simulink model "speedgoat_IO397_RCP_BLDC_openloop"  (R2025b)
settings: Solver=FixedStepDiscrete  StartTime=0.0  StopTime=inf  RelTol=1e-3
PreLoadFcn:
  | Ts = 0.001;
  | FPGA_Frequency = 75000000;
InitFcn:
  | load speedgoat_IO397_RCP_OpenLoop_Initialize.mat;
values from neighbouring files (symbols this model uses):
  motor =     [speedgoat_IO397_RCP_OpenLoop_Initialize.mat]
  target =     [speedgoat_IO397_RCP_OpenLoop_Initialize.mat]
undefined symbols (not defined in the file or in its folder): bit, DiscIntNeverNeededParam, IO397, Pull, pull, up
libraries: mcbcontrolslib x4, mcbpositiondecoderlib x3, c2837xDlib x2, c2802xlib x2, speedgoatlib_fpga_dio x1, speedgoatlib_fpga_analog_io x1, speedgoatlib_fpga_pwm x1, speedgoatlib_fpga_quadrature x1, speedgoatlib_fpga x1
settings Model: SimulationMode=external  ExtModeEnableFloating=off  Creator=simon.beck  LastModifiedBy=PattarapolSangaroon
settings SolverCC: ConcurrentTasks=on  PositivePriorityOrder=on  MaxZcPerStep=1.0
settings DataIOCC: SaveFormat=StructureWithTime
settings OptimizationCC: BlockReduction=off  OptimizeBlockIOStorage=off  BufferReuse=off  ReuseModelBlockBuffer=off
settings DebuggingCC: UnderspecifiedInitializationDetection=Classic  MergeDetectMultiDrivingBlocksExec=none  TasksWithSamePriorityMsg=none
settings HardwareCC: ProdBitPerLong=64.0  ProdLongLongMode=on  ProdHWDeviceType=Intel->x86-64 (Linux 64)
settings ModelReferenceCC: EnableRefExpFcnMdlSchedulingChecks=on  PropagateSignalLabelsOutOfModel=off
settings RTWCC: SystemTargetFile=speedgoat.tlc  TemplateMakefile=slrealtime_default_tmf  Toolchain=Simulink Real-Time Toolchain  BuildConfiguration=Faster Runs  CodeExecutionProfiling=on  TargetLang=C++  GPUComputeCapability=3.5  DLArmComputeVersion=19.05  Description=Speedgoat Real-Time Target Machine
settings SimulinkRealTimeTargetCC: SLRTFileLogMaxRuns=1.0  ExtModeMaxTrigDuration=10.0  ExtModeStaticAllocSize=1000000.0  ExtModeTransport=0.0  MultiwordLength=2048.0  DynamicStringBufferSize=256.0  PreserveMATLABNamespacesInGeneratedCode=on  SubcomponentCodeInterfacePackaging=Reusable function  InstructionSetFMA=off  LogToMDFFile=off

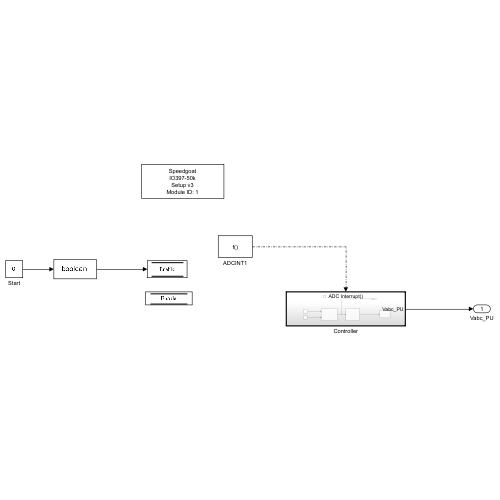
[thumbnail: Simulink's stored preview of the top-level diagram]
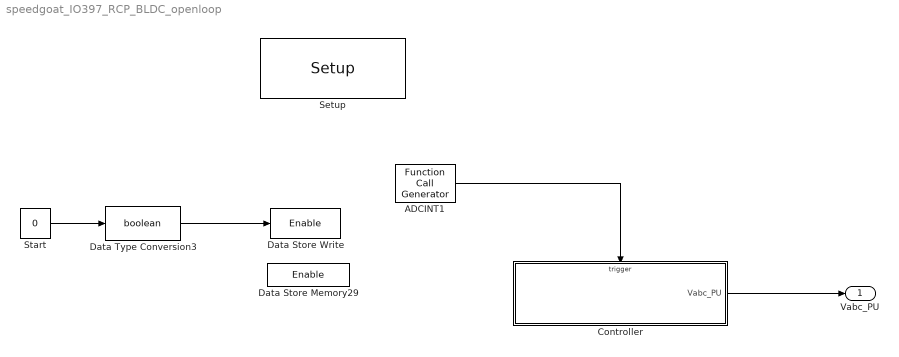
== system speedgoat_IO397_RCP_BLDC_openloop ==
  ADCINT1 : FunctionCallGenerator  SampleTime=Ts
  Controller : Subsystem
  Data Store Memory29 : DataStoreMemory  DataStoreName=Enable  ShowAdditionalParam=off  OutDataTypeStr=boolean
  Data Store Write : DataStoreWrite  DataStoreName=Enable  IndexOptions=Index vector (dialog)  Indices=1  OutputSizes=1
  Data Type Conversion3 : DataTypeConversion  OutDataTypeStr=boolean  RndMeth=Simplest  SaturateOnIntegerOverflow=off
  Setup : speedgoatlib_fpga/Setup/Setup  board=IO397-50k  id=1  pciSlot=-1  device_id=1  bitstreamFilePath=C:\ProgramData\Speedgoat\bitstreams\io_configuration_package\R2025b\io397  bitstreamFile=speedgoat_IO397_RCP.mat  fpgaFreq=75000000  enableDma=off  rearEnb_1=off  rearIO_1=None  rearEnb_2=off  rearIO_2=None  ProgSpiFlash=off  ProgBPIFlash=off  useFpgaDmaController=off  dmaStopOnOverload=on  dmaModeSequential=on  dmaModeParallel=off  dmaTrigFixTime=on  dmaTrigA2B=off  dmaTriggerSourceSel=0  PullRPort15=pull-up 3.3V  PullRPort31=pull-up 3.3V  PullRPort47=pull-up 3.3V  PullRPort63=pull-up 3.3V  diffLineTermination_1=on  diffLineTermination_2=on  diffLineTermination_3=on  diffLineTermination_4=on  diffLineTermination_5=on  diffLineTermination_6=on  diffLineTermination_7=on  diffLineTermination_8=on  diffLineTermination_9=on  diffLineTermination_10=on  diffLineTermination_11=on  diffLineTermination_12=on  diffLineTermination_13=on  diffLineTermination_14=on  diffLineTermination_15=on  diffLineTermination_16=on  diffLineTermination_17=on  diffLineTermination_18=on  diffLineTermination_19=on  diffLineTermination_20=on  diffLineTermination_21=on  diffLineTermination_22=on  diffLineTermination_23=on  diffLineTermination_24=on  diffLineTermination_25=on  diffLineTermination_26=on  diffLineTermination_27=on  diffLineTermination_28=on  diffLineTermination_29=on  diffLineTermination_30=on  diffLineTermination_31=on  diffLineTermination_32=on  ioVoltageDropDown1=3.3V  pullResistorDropDown1_1=Pull-up  pullResistorDropDown1_2=Pull-up  pullResistorDropDown1_3=Pull-up  pullResistorDropDown1_4=Pull-up  pullResistorDropDown1_5=Pull-up  pullResistorDropDown1_6=Pull-up  pullResistorDropDown1_7=Pull-up  pullResistorDropDown1_8=Pull-up  ttlIsImplementedCheckBox1=off  pullResistorDropDown2=Pull-up  ioVoltageDropDown2=3.3V  ttlIsImplementedCheckBox2=off  pullResistorDropDown3=Pull-up  ioVoltageDropDown3=3.3V  ttlIsImplementedCheckBox3=off  pullResistorDropDown4=Pull-up  ioVoltageDropDown4=3.3V  ttlIsImplementedCheckBox4=off  pullResistorDropDown5=Pull-up  ioVoltageDropDown5=3.3V  ttlIsImplementedCheckBox5=off  pullResistorDropDown6=Pull-up  ioVoltageDropDown6=3.3V  ttlIsImplementedCheckBox6=off  pullResistorDropDown7=Pull-up  ioVoltageDropDown7=3.3V  ttlIsImplementedCheckBox7=off  pullResistorDropDown8=Pull-up  ioVoltageDropDown8=3.3V  ttlIsImplementedCheckBox8=off  terminationCheckBox1=off  terminationCheckBox2=off  terminationCheckBox3=off  terminationCheckBox4=off  diffIsImplementedCheckBox1=off  terminationCheckBox5=off  terminationCheckBox6=off  terminationCheckBox7=off  terminationCheckBox8=off  diffIsImplementedCheckBox2=off  terminationCheckBox9=off  terminationCheckBox10=off  terminationCheckBox11=off  terminationCheckBox12=off  diffIsImplementedCheckBox3=off  terminationCheckBox13=off  terminationCheckBox14=off  terminationCheckBox15=off  terminationCheckBox16=off  diffIsImplementedCheckBox4=off  terminationCheckBox17=off  terminationCheckBox18=off  terminationCheckBox19=off  terminationCheckBox20=off  diffIsImplementedCheckBox5=off  terminationCheckBox21=off  terminationCheckBox22=off  terminationCheckBox23=off  terminationCheckBox24=off  diffIsImplementedCheckBox6=off  terminationCheckBox25=off  terminationCheckBox26=off  terminationCheckBox27=off  terminationCheckBox28=off  diffIsImplementedCheckBox7=off  terminationCheckBox29=off  terminationCheckBox30=off  terminationCheckBox31=off  terminationCheckBox32=off  diffIsImplementedCheckBox8=off  PullRPort0_1=pull-up  VioPort0_1=3.3V  PullRPort1_1=pull-up  VioPort1_1=3.3V  PullRPort2_1=pull-up  VioPort2_1=3.3V  PullRPort3_1=pull-up  VioPort3_1=3.3V  PullRPort4_1=pull-up  VioPort4_1=3.3V  PullRPort5_1=pull-up  VioPort5_1=3.3V  PullRPort6_1=pull-up  VioPort6_1=3.3V  diffLineTermination_rear1_1=on  diffLineTermination_rear1_2=on  diffLineTermination_rear1_3=on  diffLineTermination_rear1_4=on  diffLineTermination_rear1_5=on  diffLineTermination_rear1_6=on  diffLineTermination_rear1_7=on  diffLineTermination_rear1_8=on  PullRPort0_2=pull-up  VioPort0_2=3.3V  PullRPort1_2=pull-up  VioPort1_2=3.3V  PullRPort2_2=pull-up  VioPort2_2=3.3V  PullRPort3_2=pull-up  VioPort3_2=3.3V  PullRPort4_2=pull-up  VioPort4_2=3.3V  PullRPort5_2=pull-up  VioPort5_2=3.3V  PullRPort6_2=pull-up  VioPort6_2=3.3V  diffLineTermination_rear2_1=on  diffLineTermination_rear2_2=on  diffLineTermination_rear2_3=on  diffLineTermination_rear2_4=on  diffLineTermination_rear2_5=on  diffLineTermination_rear2_6=on  diffLineTermination_rear2_7=on  diffLineTermination_rear2_8=on
      settings: SourceProductName=IO3xx
  Start : Constant  Value=0  OutDataTypeStr=Inherit: Inherit via back propagation
  Vabc_PU : Outport  VectorParamsAs1DForOutWhenUnconnected=off
  wires:
  Data Type Conversion3/1 -> Data Store Write/1
  Start/1 -> Data Type Conversion3/1
  Controller/1(Vabc_PU) -> Vabc_PU/1
  ADCINT1/1 -> Controller/Trigger

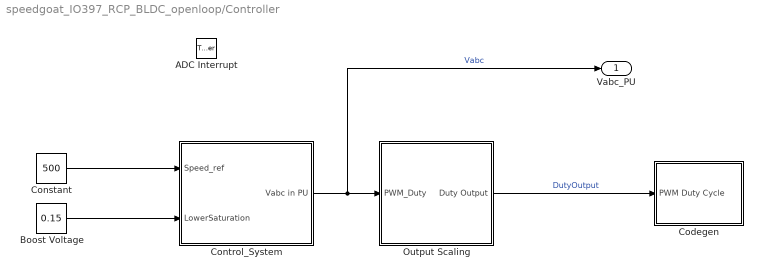
== system speedgoat_IO397_RCP_BLDC_openloop/Controller ==
  ADC Interrupt : TriggerPort  TriggerType=function-call  VariantControl=(inherit)
  Boost Voltage : Constant  Value=0.15  OutDataTypeStr=Inherit: Inherit via back propagation
  Codegen : Subsystem  VariantControl=(codegen)
  Constant : Constant  Value=500  OutDataTypeStr=Inherit: Inherit via back propagation
  Control_System : Subsystem
  Output Scaling : Subsystem
  Vabc_PU : Outport  VectorParamsAs1DForOutWhenUnconnected=off
  wires:
  Boost Voltage/1 -> Control_System/2(LowerSaturation)
  Control_System/1(Vabc in PU) -> Vabc_PU/1, Output Scaling/1(PWM_Duty)  "Vabc"
  Constant/1 -> Control_System/1(Speed_ref)
  Output Scaling/1(Duty Output) -> Codegen/1(PWM Duty Cycle)  "DutyOutput"

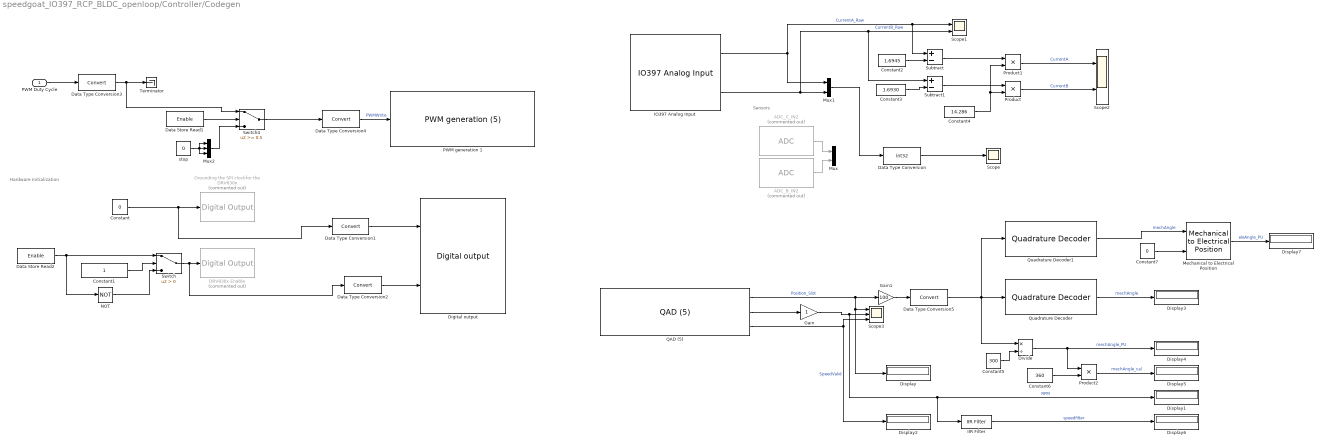
== system speedgoat_IO397_RCP_BLDC_openloop/Controller/Codegen ==
  note: Sensors
  note: Hardware Initialization
  PWM Duty Cycle : Inport
  " Grounding the SPI clockfor the DRV830x" : c2837xDlib/Digital Output  Commented=on  GPIO_Number=GPIO56~GPIO63  GPIO_Bit0=off  GPIO_BIT0_Toggle=off  GPIO_Bit1=off  GPIO_BIT1_Toggle=off  GPIO_Bit2=off  GPIO_BIT2_Toggle=off  GPIO_Bit3=off  GPIO_BIT3_Toggle=off  GPIO_Bit4=on  GPIO_BIT4_Toggle=off  GPIO_Bit5=off  GPIO_BIT5_Toggle=off  GPIO_Bit6=off  GPIO_BIT6_Toggle=off  GPIO_Bit7=off  GPIO_BIT7_Toggle=off
  ADC_B_IN2 : c2802xlib/ADC  Commented=on  blkParamProc=C2000_Type4  ADCModule=B  samplingMode=Single sample mode  ADCResolution=12-bit (Single-ended input)  ADC29xResolution=12-bit  ADCMode=Single-ended input  useSOC1=SOC0  useSOC2=SOC0_SOC1  SOCAcquisitionWindow=15  SOCTriggerSource=ePWM1_ADCSOCA  SOCInterruptTrigger=No ADCINT  Ts=-1  dType=uint16  postInterrupt=on  interruptSel=ADCINT1  ADCINTContinuous=on  endma=off  chdma=1  conv1=ADCINA0  conv2=ADCINA0 and ADCINB0  conv1_Type4=ADCIN2  conv2_Type4=ADCIN0 and ADCIN1
  ADC_C_IN2 : c2802xlib/ADC  Commented=on  blkParamProc=C2000_Type4  ADCModule=C  samplingMode=Single sample mode  ADCResolution=12-bit (Single-ended input)  ADC29xResolution=12-bit  ADCMode=Single-ended input  useSOC1=SOC0  useSOC2=SOC0_SOC1  SOCAcquisitionWindow=15  SOCTriggerSource=ePWM1_ADCSOCA  SOCInterruptTrigger=No ADCINT  Ts=-1  dType=uint16  postInterrupt=off  interruptSel=ADCINT1  ADCINTContinuous=on  endma=off  chdma=1  conv1=ADCINA0  conv2=ADCINA0 and ADCINB0  conv1_Type4=ADCIN2  conv2_Type4=ADCIN0 and ADCIN1
  Constant : Constant  Value=0  OutDataTypeStr=uint16  SampleTime=-1
  Constant1 : Constant  OutDataTypeStr=uint16
  Constant2 : Constant  Value=1.6945
  Constant3 : Constant  Value=1.6930
  Constant4 : Constant  Value=14.286
  Constant5 : Constant  Value=300
  Constant6 : Constant  Value=360
  Constant7 : Constant  Value=0
  DRV830x Enable : c2837xDlib/Digital Output  Commented=on  GPIO_Number=GPIO120~GPIO127  GPIO_Bit0=off  GPIO_BIT0_Toggle=off  GPIO_Bit1=off  GPIO_BIT1_Toggle=off  GPIO_Bit2=off  GPIO_BIT2_Toggle=off  GPIO_Bit3=off  GPIO_BIT3_Toggle=off  GPIO_Bit4=on  GPIO_BIT4_Toggle=off  GPIO_Bit5=off  GPIO_BIT5_Toggle=off  GPIO_Bit6=off  GPIO_BIT6_Toggle=off  GPIO_Bit7=off  GPIO_BIT7_Toggle=off
  Data Store Read1 : DataStoreRead  DataStoreName=Enable  IndexOptions=Index vector (dialog)  Indices=1  OutputSizes=1
  Data Store Read2 : DataStoreRead  DataStoreName=Enable  IndexOptions=Index vector (dialog)  Indices=1  OutputSizes=1
  Data Type Conversion : DataTypeConversion  OutDataTypeStr=int32  ConvertRealWorld=Stored Integer (SI)  SaturateOnIntegerOverflow=off  RndMeth=Floor
  Data Type Conversion{1..5} (5 alike) : DataTypeConversion  SaturateOnIntegerOverflow=off  RndMeth=Floor
  Digital output : speedgoatlib_fpga_dio/Digital output  id=1  chan=[11,12]  init=[0]  reset=[0]  ts=-1  vectorizeInput=off
      settings: SourceProductName=Digital
  Display{,1..7} (8 alike) : Display
  Divide : Product  Inputs=*/
  Gain : Gain
  Gain1 : Gain  Gain=100
  IIR Filter : mcbcontrolslib/IIR Filter  VariantControl=Low Pass Filter  VariantSelect=Low-pass  FilterConstantInputType=Specify via dialog  Filter_constant=0.1  InitialOutput=Specify via dialog  InitialOutputValue=0  ExternalReset=none  advancedSettings=off  Ts=50e-6  cutOff_freq=353.6777
  IO397 Analog Input : speedgoatlib_fpga_analog_io/IO397/IO397 Analog Input  openMaskCallback=0  id=1  chan=[1:2]  range=+-5 V  parAiTriggerMode=I/O Module Clock  parAiInternalSignal=None  parAiDioTriggerChannel=1  parAiSampleRate=0  trigger=Initiator  ts=-1
      settings: SourceProductName=Analog IO
  Mechanical to Electrical Position : mcbpositiondecoderlib/Mechanical to Electrical Position  PolePairsInputType=Specify via dialog  NrPP=3  selectedRange=Per unit  MechOfstInputType=Input port  mechOffsetIn=0  maxAngleIn=1  InputDataType=double  VariantSelect=floating-point
  Mux : Mux  Inputs=2
  Mux1 : Mux  Inputs=2
  Mux2 : Mux  Inputs=3
  NOT : Logic  Operator=NOT  IconShape=distinctive  AllPortsSameDT=off  OutDataTypeStr=boolean
  PWM generation 1 : speedgoatlib_fpga_pwm/PWM generation (5)  id=1  chan=[1:3]  board=IO397-50k  ts=-1  pciSlot=[-1,-1]  delay=0  symmetric=Symmetric - PWM generation is centered around half the period  b_is_complement_of_a=The complement of PWM A output  deadband=[0.0]  period=[5e-5]  frequency=20000  ticks=3749  a_on=[0]  a_off=[0.000025]  pwm_a_dc=[0.0]  b_on=[0]  b_off=[0.000025]  pwm_b_dc=[0]  c_on=[0.0]  c_off=[0.0]  protection=Disabled: A and B can be high at the same moment  enable_latch_half_period=off  pwm_update=At period starts  bit_width_pwm_gen=24  trigger_duration=[100e-6]  trigger_period_start=on  trigger_half_of_the_period=off  trigger_a_on=off  trigger_a_off=off  trigger_b_on=off  trigger_b_off=off  show_a_input=on  show_b_input=off  show_c_input=off  show_period_input=off  show_force_stop_input=off  idle_a=Low when PWM generation is halted  idle_b=Low when PWM generation is halted  idle_c=Low when PWM generation is halted  cancels_pwm_generation=on  invert_a=off  invert_b=off  invert_c=off
      settings: SourceProductName=PWM
  Product : Product
  Product1 : Product
  Product2 : Product
  QAD (5) : speedgoatlib_fpga_quadrature/QAD (5)  id=1  chan=[1]  sampleTime=-1  numOfSlots=3  sensorType=Capture A + B Signal  interpolatePosition=off  swapAB=off  indexControlMode=Ignore Index  latchMode=Disabled  gateIndex=No Gating  speedFilterWidth=4  showInputSpeedFilterWidth=off  glitchFilterSeconds=106.7e-9  glitchFilterSecondsEff=106.7e-9  showInputClearPosition=off  showInputClearIndexFound=off  showOutputPosition=on  showOutputTurn=off  showOutputSpeed=on  showOutputIndexFound=off  showOutputLastPulse=off
      settings: SourceProductName=Quadrature
  Quadrature Decoder : mcbpositiondecoderlib/Quadrature Decoder  ParameterInputType=off  CountsPerRevInverseDataType=single  EncoderSlitsPerRevolution=300  EncoderCountsPerSlit=1  CounterSize=16 bits  ExternalIndexCount=off  PositionUnit=Degrees  PositionDataType=double
  Quadrature Decoder1 : mcbpositiondecoderlib/Quadrature Decoder  ParameterInputType=off  CountsPerRevInverseDataType=single  EncoderSlitsPerRevolution=300  EncoderCountsPerSlit=1  CounterSize=16 bits  ExternalIndexCount=off  PositionUnit=Per unit  PositionDataType=double
  Scope : Scope
      settings: DataLoggingVariableName=ScopeData2
  Scope1 : Scope  NumInputPorts=2
      settings: ActiveDisplayYMinimum=1.681976843626785  ActiveDisplayYMaximum=1.7058195201071538
  Scope2 : Scope  NumInputPorts=2
      settings: ActiveDisplayYMinimum=1.681976843626785  ActiveDisplayYMaximum=1.7058195201071538
  Scope3 : Scope  NumInputPorts=3
      settings: ActiveDisplayYMinimum=-0.34374999999999994  ActiveDisplayYMaximum=3.09375  DataLoggingVariableName=ScopeData3
  Subtract : Sum  Inputs=+-
  Subtract1 : Sum  Inputs=+-
  Switch : Switch  Criteria=u2 > Threshold  OutDataTypeStr=boolean  RndMeth=Simplest  SaturateOnIntegerOverflow=off  InputSameDT=off
  Switch4 : Switch  Threshold=0.5  RndMeth=Simplest  SaturateOnIntegerOverflow=off  InputSameDT=off
  Terminator : Terminator
  stop : Constant  Value=0  OutDataTypeStr=single
  wires:
  Data Type Conversion1/1 -> Digital output/1
  Data Store Read1/1 -> Switch4/2
  Mux2/1 -> Switch4/3
  stop/1 -> Mux2/3, Mux2/2, Mux2/1
  Switch4/1 -> Data Type Conversion4/1
  Data Type Conversion3/1 -> Switch4/1, Terminator/1
  ADC_C_IN2/1 -> Mux/1
  ADC_B_IN2/1 -> Mux/2
  Data Type Conversion2/1 -> Digital output/2
  Mux1/1 -> Data Type Conversion/1
  IO397 Analog Input/1 -> Subtract/1, Scope1/1, Mux1/1  "CurrentA_Raw"
  IO397 Analog Input/2 -> Subtract1/1, Scope1/2, Mux1/2  "CurrentB_Raw"
  Constant1/1 -> Switch/2
  NOT/1 -> Switch/3
  Data Type Conversion/1 -> Scope/1
  Data Store Read2/1 -> NOT/1, Switch/1
  Switch/1 -> Data Type Conversion2/1, DRV830x Enable/1
  Constant/1 -> Data Type Conversion1/1, " Grounding the SPI clockfor the DRV830x"/1
  PWM Duty Cycle/1 -> Data Type Conversion3/1
  Data Type Conversion4/1 -> PWM generation 1/1  "PWMWrite"
  Constant2/1 -> Subtract/2
  Constant3/1 -> Subtract1/2
  Subtract1/1 -> Product/1
  Subtract/1 -> Product1/1
  Constant4/1 -> Product/2, Product1/2
  Product/1 -> Scope2/2  "CurrentB"
  Product1/1 -> Scope2/1  "CurrentA"
  QAD (5)/3 -> Display2/1, Scope3/3  "SpeedValid"
  Gain/1 -> IIR Filter/1, Display1/1, Scope3/2  "RPM"
  QAD (5)/2 -> Gain/1
  QAD (5)/1 -> Gain1/1, Display/1, Scope3/1  "Position_Slot"
  Quadrature Decoder/1 -> Display3/1  "mechAngle"
  Constant5/1 -> Divide/2
  Divide/1 -> Display4/1, Product2/1  "mechAngle_PU"
  Constant6/1 -> Product2/2
  Product2/1 -> Display5/1  "mechAngle_cal"
  Data Type Conversion5/1 -> Quadrature Decoder1/1, Divide/1, Quadrature Decoder/1
  Gain1/1 -> Data Type Conversion5/1
  IIR Filter/1 -> Display6/1  "speedfilter"
  Constant7/1 -> Mechanical to Electrical Position/2
  Mechanical to Electrical Position/1 -> Display7/1  "eleAngle_PU"
  Quadrature Decoder1/1 -> Mechanical to Electrical Position/1  "mechAngle"

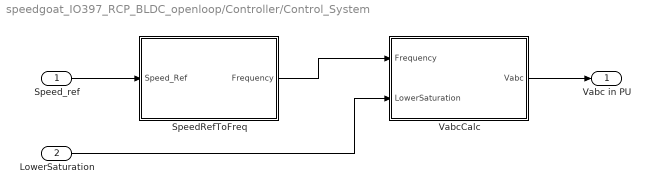
== system speedgoat_IO397_RCP_BLDC_openloop/Controller/Control_System ==
  Speed_ref : Inport
  LowerSaturation : Inport  Port=2
  SpeedRefToFreq : Subsystem
  VabcCalc : Subsystem
  Vabc in PU : Outport  VectorParamsAs1DForOutWhenUnconnected=off
  wires:
  Speed_ref/1 -> SpeedRefToFreq/1(Speed_Ref)
  SpeedRefToFreq/1(Frequency) -> VabcCalc/1(Frequency)
  VabcCalc/1(Vabc) -> Vabc in PU/1
  LowerSaturation/1 -> VabcCalc/2(LowerSaturation)

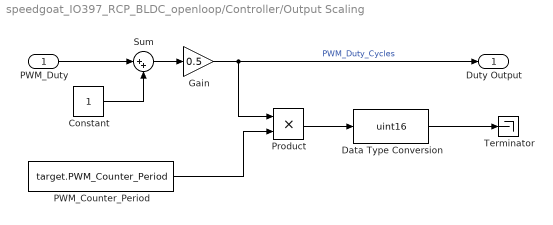
== system speedgoat_IO397_RCP_BLDC_openloop/Controller/Output Scaling ==
  PWM_Duty : Inport
  Constant : Constant  OutDataTypeStr=dataType
  Data Type Conversion : DataTypeConversion  OutDataTypeStr=uint16  RndMeth=Floor
  Gain : Gain  Gain=0.5  RndMeth=Simplest  OutDataTypeStr=Inherit: Same as input
  PWM_Counter_Period : Constant  Value=target.PWM_Counter_Period  OutDataTypeStr=dataType  SampleTime=-1
  Product : Product  RndMeth=Simplest  OutDataTypeStr=Inherit: Same as first input
  Sum : Sum  Inputs=|++
  Terminator : Terminator
  Duty Output : Outport
  wires:
  PWM_Counter_Period/1 -> Product/2
  PWM_Duty/1 -> Sum/1
  Product/1 -> Data Type Conversion/1
  Constant/1 -> Sum/2
  Sum/1 -> Gain/1
  Gain/1 -> Duty Output/1, Product/1  "PWM_Duty_Cycles"
  Data Type Conversion/1 -> Terminator/1

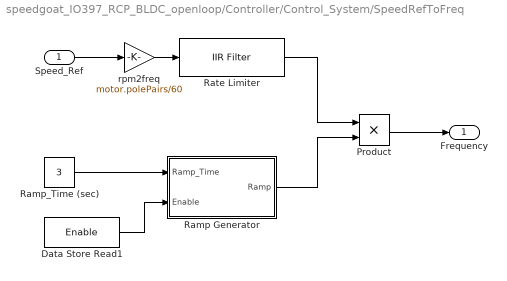
== system speedgoat_IO397_RCP_BLDC_openloop/Controller/Control_System/SpeedRefToFreq ==
  Speed_Ref : Inport
  Data Store Read1 : DataStoreRead  DataStoreName=Enable  IndexOptions=Index vector (dialog)  Indices=1  OutputSizes=1
  Product : Product  RndMeth=Simplest  OutDataTypeStr=Inherit: Same as first input
  Ramp Generator : Subsystem
  Ramp_Time (sec) : Constant  Value=3  SampleTime=-1
  Rate Limiter : mcbcontrolslib/IIR Filter  VariantControl=Low Pass Filter  VariantSelect=Low-pass  FilterConstantInputType=Specify via dialog  Filter_constant=0.0001  InitialOutput=Specify via dialog  InitialOutputValue=0  ExternalReset=none  advancedSettings=off  Ts=50e-6  cutOff_freq=0.31834
  rpm2freq : Gain  Gain=motor.polePairs/60  OutDataTypeStr=dataType  RndMeth=Simplest
  Frequency : Outport
  wires:
  Product/1 -> Frequency/1
  Ramp Generator/1(Ramp) -> Product/2
  Ramp_Time (sec)/1 -> Ramp Generator/1(Ramp_Time)
  rpm2freq/1 -> Rate Limiter/1
  Data Store Read1/1 -> Ramp Generator/2(Enable)
  Speed_Ref/1 -> rpm2freq/1
  Rate Limiter/1 -> Product/1

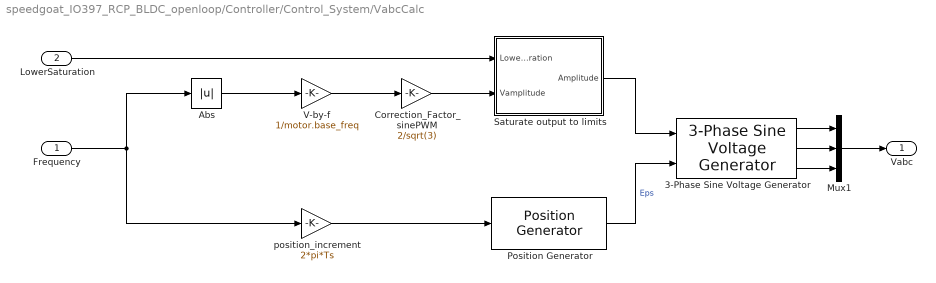
== system speedgoat_IO397_RCP_BLDC_openloop/Controller/Control_System/VabcCalc ==
  Frequency : Inport
  LowerSaturation : Inport  Port=2
  3-Phase Sine Voltage Generator : mcbcontrolslib/3-Phase Sine Voltage Generator  AngleInput=Radians  N_points=1024
  Abs : Abs  RndMeth=Simplest  SaturateOnIntegerOverflow=off
  Correction_Factor_sinePWM : Gain  Gain=2/sqrt(3)  RndMeth=Simplest  OutDataTypeStr=Inherit: Same as input
  Mux1 : Mux  Inputs=3
  Position Generator : mcbcontrolslib/Position Generator  AngleOutput=Radians  InitialThetaSource=Specify via dialog  ExternalReset=none  Offset=0
  Saturate output to limits : Subsystem
  V-by-f : Gain  Gain=1/motor.base_freq  RndMeth=Simplest  OutDataTypeStr=Inherit: Same as input
  position_increment : Gain  Gain=2*pi*Ts  RndMeth=Simplest  OutDataTypeStr=Inherit: Same as input
  Vabc : Outport
  wires:
  Frequency/1 -> Abs/1, position_increment/1
  position_increment/1 -> Position Generator/1
  3-Phase Sine Voltage Generator/3 -> Mux1/3
  3-Phase Sine Voltage Generator/2 -> Mux1/2
  V-by-f/1 -> Correction_Factor_sinePWM/1
  3-Phase Sine Voltage Generator/1 -> Mux1/1
  Correction_Factor_sinePWM/1 -> Saturate output to limits/2(Vamplitude)
  Mux1/1 -> Vabc/1
  LowerSaturation/1 -> Saturate output to limits/1(Lower Saturation)
  Saturate output to limits/1(Amplitude) -> 3-Phase Sine Voltage Generator/1
  Position Generator/1 -> 3-Phase Sine Voltage Generator/2  "Eps"
  Abs/1 -> V-by-f/1

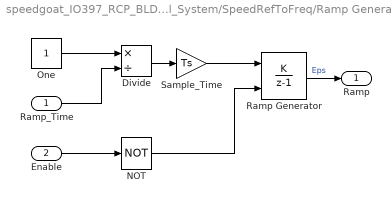
== system speedgoat_IO397_RCP_BLDC_openloop/Controller/Control_System/SpeedRefToFreq/Ramp Generator ==
  Ramp_Time : Inport
  Enable : Inport  Port=2
  Divide : Product  Inputs=*/  RndMeth=Simplest  OutDataTypeStr=Inherit: Same as first input
  NOT : Logic  Operator=NOT  IconShape=distinctive  AllPortsSameDT=off  OutDataTypeStr=boolean
  One : Constant  SampleTime=-1
  Ramp Generator : DiscreteIntegrator  IntegratorMethod=Accumulation: Forward Euler  gainval=1  ExternalReset=sampled level  SampleTime=-1  OutDataTypeStr=dataType  RndMeth=Simplest  LimitOutput=on  UpperSaturationLimit=1  LowerSaturationLimit=0  ICPrevOutput=DiscIntNeverNeededParam  ICPrevScaledInput=DiscIntNeverNeededParam
  Sample_Time : Gain  Gain=Ts  RndMeth=Simplest  OutDataTypeStr=Inherit: Same as input
  Ramp : Outport
  wires:
  Divide/1 -> Sample_Time/1
  Ramp Generator/1 -> Ramp/1  "Eps"
  Sample_Time/1 -> Ramp Generator/1
  One/1 -> Divide/1
  Ramp_Time/1 -> Divide/2
  Enable/1 -> NOT/1
  NOT/1 -> Ramp Generator/2

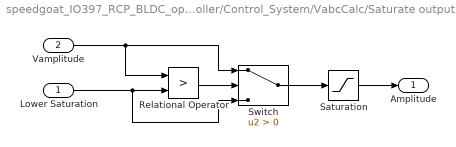
== system speedgoat_IO397_RCP_BLDC_openloop/Controller/Control_System/VabcCalc/Saturate output to limits ==
  Lower Saturation : Inport
  Vamplitude : Inport  Port=2
  Relational Operator : RelationalOperator  Operator=>  OutDataTypeStr=boolean  RndMeth=Simplest  InputSameDT=off
  Saturation : Saturate  UpperLimit=0.95  LowerLimit=0  RndMeth=Simplest
  Switch : Switch  Criteria=u2 > Threshold  SaturateOnIntegerOverflow=off  InputSameDT=off
  Amplitude : Outport
  wires:
  Saturation/1 -> Amplitude/1
  Switch/1 -> Saturation/1
  Relational Operator/1 -> Switch/2
  Lower Saturation/1 -> Switch/3, Relational Operator/2
  Vamplitude/1 -> Switch/1, Relational Operator/1
